simulink model "mit_ctl"  (R2023a)
settings: configuration reference "config" (kept outside this file)
libraries: simulink x1
settings Model: DataDictionary=model_config.sldd  Creator=huangcheng  LastModifiedBy=Administrator
settings ConfigSetRef: SourceName=config

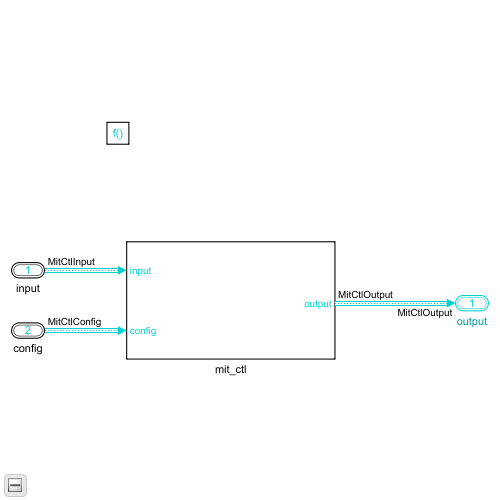
[thumbnail: Simulink's stored preview of the top-level diagram]
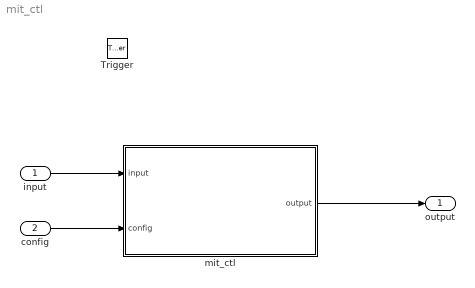
== system mit_ctl ==
  input : Inport  OutDataTypeStr=Bus: MitCtlInput  BusOutputAsStruct=on
  config : Inport  Port=2  OutDataTypeStr=Bus: MitCtlConfig  BusOutputAsStruct=on
  Trigger : TriggerPort  TriggerType=function-call  VariantControl=(inherit)  PortDimensions=1
  mit_ctl : Subsystem
  output : Outport  OutDataTypeStr=Bus: MitCtlOutput  BusOutputAsStruct=on
  wires:
  input/1 -> mit_ctl/1(input)
  config/1 -> mit_ctl/2(config)
  mit_ctl/1(output) -> output/1

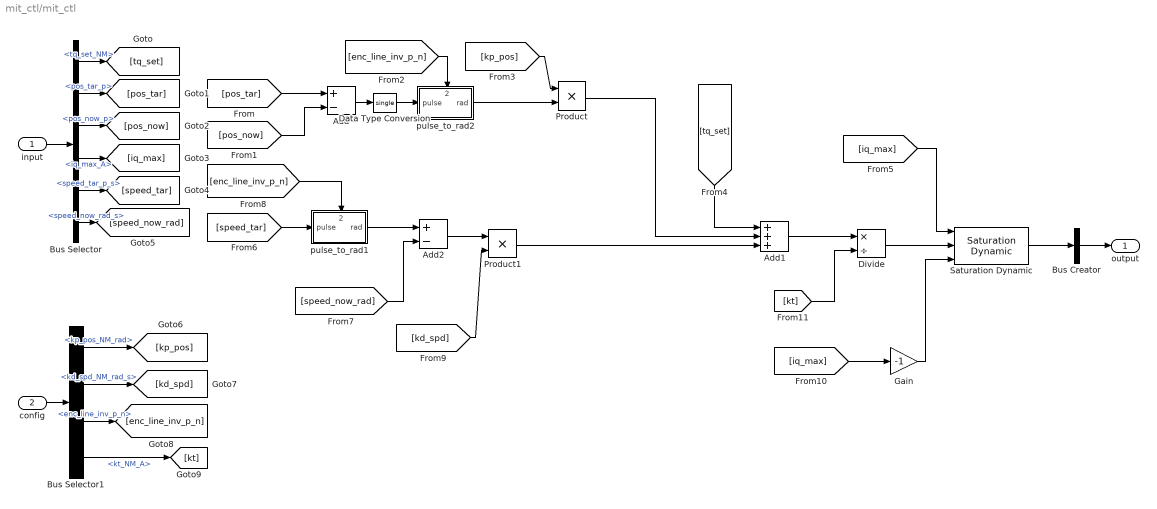
== system mit_ctl/mit_ctl ==
  input : Inport  OutDataTypeStr=Bus: MitCtlInput
  config : Inport  Port=2  OutDataTypeStr=Bus: MitCtlConfig
  Add : Sum  Inputs=+-
  Add1 : Sum  Inputs=+++
  Add2 : Sum  Inputs=+-
  Bus Creator : BusCreator  Inputs=1  OutDataTypeStr=Bus: MitCtlOutput  NonVirtualBus=on
      settings: InheritFromInputs=off
  Bus Selector : BusSelector  OutputSignals=tq_set_NM,pos_tar_p,pos_now_p,iq_max_A,speed_tar_p_s,speed_now_rad_s
  Bus Selector1 : BusSelector  OutputSignals=kp_pos_NM_rad,kd_spd_NM_rad_s,enc_line_inv_p_n,kt_NM_A
  Data Type Conversion : DataTypeConversion  OutDataTypeStr=single  SaturateOnIntegerOverflow=off  RndMeth=Floor
  Divide : Product  Inputs=*/
  Gain : Gain  Gain=-1
  Product : Product
  Product1 : Product
  Saturation Dynamic : simulink/Discontinuities/Saturation Dynamic  OutMin=[]  OutMax=[]  OutDataTypeStr=Inherit: Same as second input  OutDataType=fixdt(1, 16)  OutScaling=2^-10  DoSatur=off
  pulse_to_rad1 : Subsystem
      settings: PortSchema="{\"entries\":[{\"content\":{\"sides\":[{\"content\":{\"connectorIds\":[\"In1\"]},\"type\":\"ConnectorPlacement.EquallySpacedRectSide\",\"uuid\":\"b4823d95-7c69-4874-b59f-7c369b0996d8\"},{\"content\":{\"connectorIds\":[\"Out1\"],\"side\":\"RIGHT\"},\"type\":\"ConnectorPlacement.EquallySpacedRectSide\",\"uuid\":\"88ca7b05-7b7a-41ee-b921-df5a41d5bc09\"},{\"content\":{\"connectorIds\":[\"In2\"],\"side\":\"TOP\"},\"type\":\"ConnectorPlacement.EquallySpacedRectSide\",\"uuid\":\"eb8dd953-0ac7-435c-b49c-a5d9a4d409fd\"}]},\"type\":\"ConnectorPlacement.EquallySpacedConnector\",\"uuid\":\"c2f956bc-4785-43dd-a735-6bde8e889993\"}],\"packageUris\":[\"http://schema.mathworks.com/mf0/Connector/R2020b\"],\"version\":\"1.0\"}"
  pulse_to_rad2 : Subsystem
      settings: PortSchema="{\"entries\":[{\"content\":{\"sides\":[{\"content\":{\"connectorIds\":[\"In1\"]},\"type\":\"ConnectorPlacement.EquallySpacedRectSide\",\"uuid\":\"b4823d95-7c69-4874-b59f-7c369b0996d8\"},{\"content\":{\"connectorIds\":[\"Out1\"],\"side\":\"RIGHT\"},\"type\":\"ConnectorPlacement.EquallySpacedRectSide\",\"uuid\":\"88ca7b05-7b7a-41ee-b921-df5a41d5bc09\"},{\"content\":{\"connectorIds\":[\"In2\"],\"side\":\"TOP\"},\"type\":\"ConnectorPlacement.EquallySpacedRectSide\",\"uuid\":\"eb8dd953-0ac7-435c-b49c-a5d9a4d409fd\"}]},\"type\":\"ConnectorPlacement.EquallySpacedConnector\",\"uuid\":\"c2f956bc-4785-43dd-a735-6bde8e889993\"}],\"packageUris\":[\"http://schema.mathworks.com/mf0/Connector/R2020b\"],\"version\":\"1.0\"}"
  output : Outport  OutDataTypeStr=Bus: MitCtlOutput
  wires:
  Bus Selector/4 -> [iq_max]  "<iq_max_A>"
  Bus Selector/3 -> [pos_now]  "<pos_now_p>"
  Bus Selector/1 -> [tq_set]  "<tq_set_NM>"
  input/1 -> Bus Selector/1
  config/1 -> Bus Selector1/1
  Bus Selector/6 -> [speed_now_rad]  "<speed_now_rad_s>"
  Bus Selector/5 -> [speed_tar]  "<speed_tar_p_s>"
  Bus Selector/2 -> [pos_tar]  "<pos_tar_p>"
  Bus Selector1/1 -> [kp_pos]  "<kp_pos_NM_rad>"
  Bus Selector1/2 -> [kd_spd]  "<kd_spd_NM_rad_s>"
  Bus Selector1/3 -> [enc_line_inv_p_n]  "<enc_line_inv_p_n>"
  [pos_tar] -> Add/1
  [pos_now] -> Add/2
  Add/1 -> Data Type Conversion/1
  [enc_line_inv_p_n] -> pulse_to_rad2/2(enc_line_inv_p_s)
  pulse_to_rad2/1(rad) -> Product/2
  [kp_pos] -> Product/1
  [tq_set] -> Add1/1
  Product/1 -> Add1/2
  [enc_line_inv_p_n] -> pulse_to_rad1/2(enc_line_inv_p_s)
  [speed_tar] -> pulse_to_rad1/1(pulse)
  pulse_to_rad1/1(rad) -> Add2/1
  [speed_now_rad] -> Add2/2
  Add2/1 -> Product1/1
  [kd_spd] -> Product1/2
  Product1/1 -> Add1/3
  [iq_max] -> Saturation Dynamic/1
  [iq_max] -> Gain/1
  Gain/1 -> Saturation Dynamic/3
  Saturation Dynamic/1 -> Bus Creator/1
  Bus Creator/1 -> output/1
  Data Type Conversion/1 -> pulse_to_rad2/1(pulse)
  Bus Selector1/4 -> [kt]  "<kt_NM_A>"
  Add1/1 -> Divide/1
  Divide/1 -> Saturation Dynamic/2
  [kt] -> Divide/2

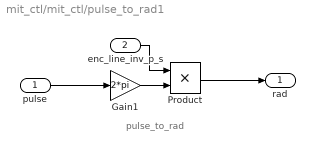
== system mit_ctl/mit_ctl/pulse_to_rad1 ==
  note: pulse_to_rad
  pulse : Inport
  enc_line_inv_p_s : Inport  Port=2
  Gain1 : Gain  Gain=2*pi
  Product : Product
  rad : Outport
  wires:
  Gain1/1 -> Product/2
  Product/1 -> rad/1
  pulse/1 -> Gain1/1
  enc_line_inv_p_s/1 -> Product/1

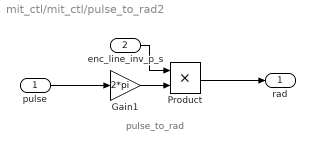
== system mit_ctl/mit_ctl/pulse_to_rad2 ==
  note: pulse_to_rad
  pulse : Inport
  enc_line_inv_p_s : Inport  Port=2
  Gain1 : Gain  Gain=2*pi
  Product : Product
  rad : Outport
  wires:
  Gain1/1 -> Product/2
  Product/1 -> rad/1
  pulse/1 -> Gain1/1
  enc_line_inv_p_s/1 -> Product/1
